simulink model "simltic"  (Simulink 8.5)
settings: Solver=ode45  StartTime=0.0  StopTime=1  RelTol=1e-3
values from neighbouring files (symbols this model uses):
  F = [0  1; -0.9  -0.8]    [harmosc_ricatti.mat]    (also in harmosc_riccati.mat; lec.m = ones(n,1); state9.m = [ 0     rho_z  -rho_y     1     0     0     0     0     0; state9_01.mat = [0 0 -7.85492378154e-07 -1.53754144823e-06 0 0 0 0 0 0 0 -7.)
  H = [1 0]    [constant_velocity.m]    (also in damposc.m; harmosc_ricatti.mat; harmosc_riccati.mat; kf_resistor_demo.m = 1)
  I = [1  0; 0  1]    [harmosc_ricatti.mat]    (also in harmosc_riccati.mat; kalgen.m = eye(n); lec.m = ones(n,1); state9.m = eye(n))
  P0 = [0.01 0; 0 0.01]    [constant_velocity.m]    (also in damposc.m; harmosc_ricatti.mat = [0.95  0; 0  1]; harmosc_riccati.mat = [1  0; 0  1]; kalgen.m = proc_noise * eye(n))
  Q = [0.0001 0; 0 0.000001]    [constant_velocity.m]    (also in damposc.m = [0.00001 0; 0 0.000001]; harmosc_ricatti.mat = [1  0; 0  1]; harmosc_riccati.mat = [1  0; 0  1]; kalgen.m = proc_noise * eye(n))
  R = Re + h    (= 6378441.8)    [Ainit.m]    (also in constant_velocity.m = 1; damposc.m = 0.01; harmosc_ricatti.mat = 2; harmosc_riccati.mat = 3)
undefined symbols (not defined in the file or in its folder): rss_ratio, ud_inv
settings Model: Creator=mcarroll  LastModifiedBy=1104070  ExtModeAutoUpdateStatusClock=off
settings DataIOCC: SaveFormat=StructureWithTime  SignalLoggingName=sigsOut
settings OptimizationCC: OptimizeBlockIOStorage=off  BufferReuse=off  GlobalBufferReuse=off  ExpressionFolding=off  LocalBlockOutputs=off
settings DebuggingCC: SaveWithParameterizedLinksMsg=none  SignalResolutionControl=TryResolveAllWithWarning  MultiTaskDSMMsg=warning  MultiTaskCondExecSysMsg=none  FcnCallInpInsideContextMsg=UseLocalSettings
settings HardwareCC: TargetUnknown=on

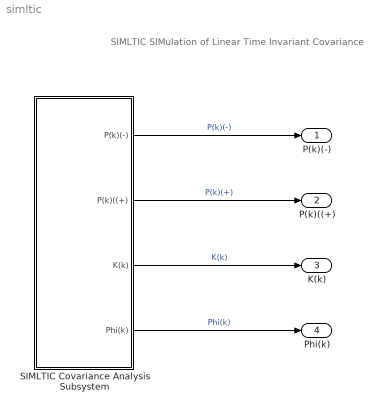
== system simltic ==
  note: SIMLTIC
      | SIMulation of Linear Time Invariant Covariance
  SIMLTIC Covariance Analysis Subsystem : Subsystem
  P(k)(-) : Outport
  P(k)((+) : Outport  Port=2
  K(k) : Outport  Port=3
  Phi(k) : Outport  Port=4
  wires:
  SIMLTIC Covariance Analysis Subsystem/1(P(k)(-)) -> P(k)(-)/1  "P(k)(-)"
  SIMLTIC Covariance Analysis Subsystem/2(P(k)((+)) -> P(k)((+)/1  "P(k)(+)"
  SIMLTIC Covariance Analysis Subsystem/3(K(k)) -> K(k)/1  "K(k)"
  SIMLTIC Covariance Analysis Subsystem/4(Phi(k)) -> Phi(k)/1  "Phi(k)"

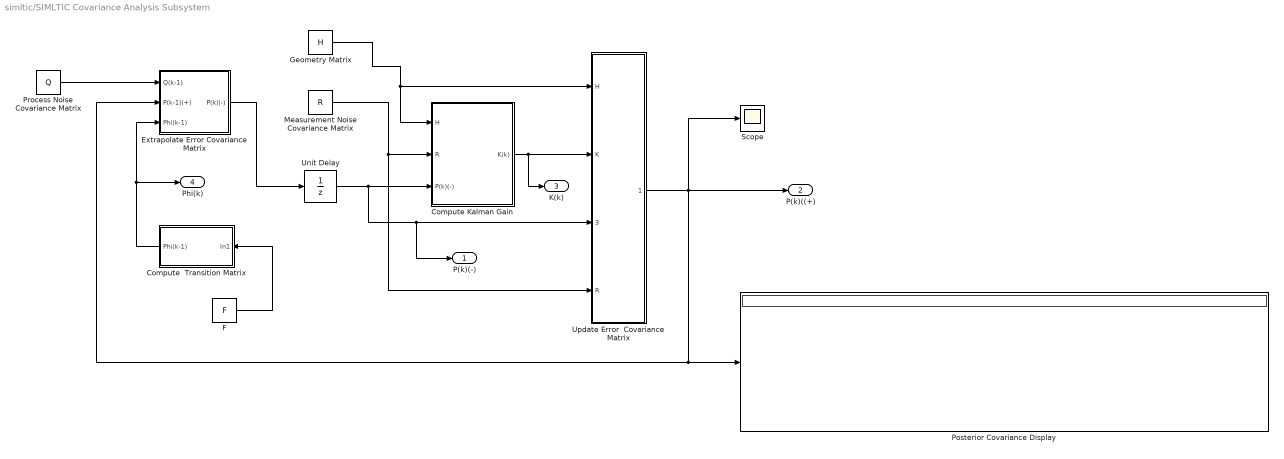
== system simltic/SIMLTIC Covariance Analysis Subsystem ==
  Compute  Transition Matrix : Subsystem
  Compute Kalman Gain : Subsystem
  Extrapolate Error Covariance Matrix : Subsystem
  F : Constant  Value=F  VectorParams1D=off
  Geometry Matrix : Constant  Value=H  VectorParams1D=off
  Measurement Noise Covariance Matrix : Constant  Value=R  VectorParams1D=off
  Posterior Covariance Display : Display
  Process Noise Covariance Matrix : Constant  Value=Q  VectorParams1D=off
  Scope : Scope
      settings: TimeRange=10  YMin=-20  YMax=120  SaveName=ScopeData4
  Unit Delay : UnitDelay  InitialCondition=P0
  Update Error  Covariance Matrix : Subsystem
  P(k)(-) : Outport
  P(k)((+) : Outport  Port=2
  K(k) : Outport  Port=3
  Phi(k) : Outport  Port=4
  wires:
  Update Error  Covariance Matrix/1(P(k)(+)) -> Extrapolate Error Covariance Matrix/2(P(k-1)(+)), Posterior Covariance Display/1, P(k)((+)/1, Scope/1
  Unit Delay/1 -> Compute Kalman Gain/3(P(k)(-)), Update Error  Covariance Matrix/3(P(k)(-)), P(k)(-)/1
  Compute Kalman Gain/1(K(k)) -> Update Error  Covariance Matrix/2(K), K(k)/1
  Process Noise Covariance Matrix/1 -> Extrapolate Error Covariance Matrix/1(Q(k-1))
  Extrapolate Error Covariance Matrix/1(P(k)(-)) -> Unit Delay/1
  Compute  Transition Matrix/1(Phi(k-1)) -> Extrapolate Error Covariance Matrix/3(Phi(k-1)), Phi(k)/1
  Geometry Matrix/1 -> Compute Kalman Gain/1(H), Update Error  Covariance Matrix/1(H)
  Measurement Noise Covariance Matrix/1 -> Compute Kalman Gain/2(R), Update Error  Covariance Matrix/4(R)
  F/1 -> Compute  Transition Matrix/1(In1)

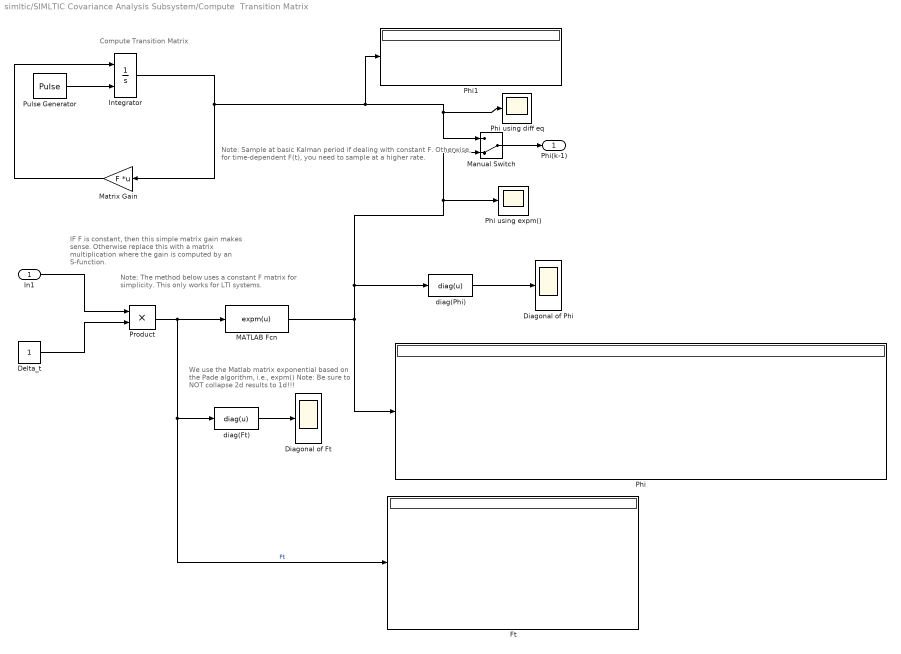
== system simltic/SIMLTIC Covariance Analysis Subsystem/Compute  Transition Matrix ==
  note: We use the Matlab matrix exponential based
      | on the Pade algorithm, i.e., expm()
      | Note:  Be sure to NOT collapse 2d results
      | to 1d!!!
  note: Note:  The method below uses a constant F matrix
      | for simplicity.  This only works for LTI
      | systems.
  note: Compute Transition Matrix
  note: Note: Sample at basic Kalman period if dealing with constant F.
      | Otherwise, for time-dependent F(t), you need to sample at a
      | higher rate.
  note: IF F is constant, then this simple
      | matrix gain makes sense.  Otherwise
      | replace this with a matrix multiplication
      | where the gain is computed by an S-function.
  In1 : Inport
  Delta_t : Constant
  Diagonal of Ft : Scope
      settings: YMin=0  YMax=2  SaveName=ScopeData18
  Diagonal of Phi : Scope
      settings: YMin=0  YMax=2  SaveName=ScopeData3
  Ft : Display
  Integrator : Integrator  ExternalReset=either  InitialCondition=I
  MATLAB Fcn : MATLABFcn  MATLABFcn=expm(u)  Output1D=off
  Manual Switch : ManualSwitch  CurrentSetting=0
  Matrix Gain : Gain  Gain=F  Multiplication=Matrix(K*u)  SaturateOnIntegerOverflow=on  OutDataTypeStr=Inherit: Same as input  ParamDataTypeStr=Inherit: Same as input
  Phi : Display
  Phi using diff eq : Scope
      settings: YMin=0  YMax=2  SaveName=ScopeData11
  Phi using expm() : Scope
      settings: YMin=0  YMax=2  SaveName=ScopeData5
  Phi1 : Display
  Product : Product  SaturateOnIntegerOverflow=on  InputSameDT=on  OutDataTypeStr=Inherit: Same as first input
  Pulse Generator : DiscretePulseGenerator  PulseType=Time based  PulseWidth=50
  diag(Ft) : MATLABFcn  MATLABFcn=diag(u)  Output1D=off
  diag(Phi) : MATLABFcn  MATLABFcn=diag(u)
  Phi(k-1) : Outport
  wires:
  Delta_t/1 -> Product/2
  diag(Ft)/1 -> Diagonal of Ft/1
  diag(Phi)/1 -> Diagonal of Phi/1
  MATLAB Fcn/1 -> Phi/1, diag(Phi)/1, Manual Switch/2, Phi using expm()/1
  Product/1 -> diag(Ft)/1, Ft/1, MATLAB Fcn/1  "Ft"
  In1/1 -> Product/1
  Integrator/1 -> Matrix Gain/1, Phi1/1, Manual Switch/1, Phi using diff eq/1
  Manual Switch/1 -> Phi(k-1)/1
  Matrix Gain/1 -> Integrator/1
  Pulse Generator/1 -> Integrator/2

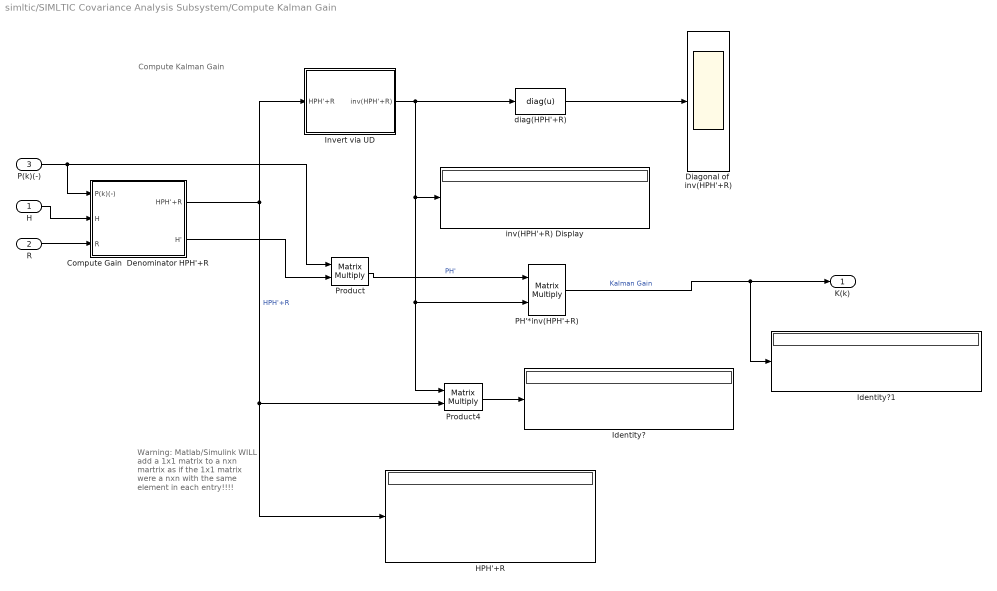
== system simltic/SIMLTIC Covariance Analysis Subsystem/Compute Kalman Gain ==
  note: Compute Kalman Gain
  note: Warning:
      | Matlab/Simulink
      | WILL add a 1x1 matrix to
      | a nxn martrix as if the
      | 1x1 matrix were a
      | nxn with the same element
      | in each entry!!!!
  H : Inport
  R : Inport  Port=2
  P(k)(-) : Inport  Port=3
  Compute Gain  Denominator HPH'+R : Subsystem
  Diagonal of  inv(HPH'+R) : Scope
      settings: TimeRange=100  YMin=0.0006  YMax=0.002  SaveName=ScopeData2
  HPH'+R : Display
  Identity? : Display
  Identity?1 : Display
  Invert via UD : Subsystem
  PH'*inv(HPH'+R) : Product  Multiplication=Matrix(*)  OutDataTypeStr=Inherit: Same as first input
  Product : Product  Multiplication=Matrix(*)  SaturateOnIntegerOverflow=on  OutDataTypeStr=Inherit: Same as first input
  Product4 : Product  Multiplication=Matrix(*)  SaturateOnIntegerOverflow=on  InputSameDT=on  OutDataTypeStr=Inherit: Same as first input
  diag(HPH'+R) : MATLABFcn  MATLABFcn=diag(u)
  inv(HPH'+R) Display : Display
  K(k) : Outport
  wires:
  Compute Gain  Denominator HPH'+R/1(HPH'+R) -> Invert via UD/1(HPH'+R), HPH'+R/1, Product4/2  "HPH'+R"
  R/1 -> Compute Gain  Denominator HPH'+R/3(R)
  diag(HPH'+R)/1 -> Diagonal of  inv(HPH'+R)/1
  Invert via UD/1(inv(HPH'+R)) -> diag(HPH'+R)/1, inv(HPH'+R) Display/1, PH'*inv(HPH'+R)/2, Product4/1
  Compute Gain  Denominator HPH'+R/2(H') -> Product/2
  Product/1 -> PH'*inv(HPH'+R)/1  "PH'"
  Product4/1 -> Identity?/1
  H/1 -> Compute Gain  Denominator HPH'+R/2(H)
  P(k)(-)/1 -> Compute Gain  Denominator HPH'+R/1(P(k)(-)), Product/1
  PH'*inv(HPH'+R)/1 -> K(k)/1, Identity?1/1  "Kalman Gain"

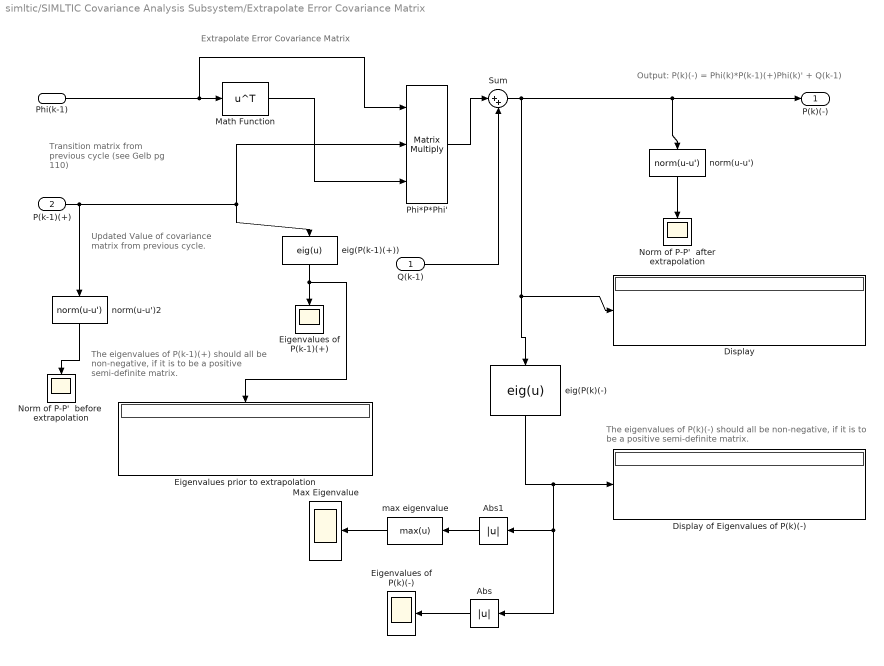
== system simltic/SIMLTIC Covariance Analysis Subsystem/Extrapolate Error Covariance Matrix ==
  note: The eigenvalues of P(k)(-) should all be non-negative,
      | if it is to be a positive semi-definite matrix.
  note: The eigenvalues of P(k-1)(+) should all be
      | non-negative, if it is to be a positive
      | semi-definite matrix.
  note: Transition matrix from
      | previous cycle
      | (see Gelb pg 110)
  note: Output: P(k)(-) = Phi(k)*P(k-1)(+)Phi(k)' + Q(k-1)
  note: Updated Value of
      | covariance matrix  from
      | previous cycle.
  note: Extrapolate Error Covariance Matrix
  Q(k-1) : Inport
  P(k-1)(+) : Inport  Port=2
  Phi(k-1) : Inport  Port=3
  Abs : Abs  SaturateOnIntegerOverflow=on
  Abs1 : Abs  SaturateOnIntegerOverflow=on
  Display : Display
  Display of Eigenvalues of P(k)(-) : Display
  Eigenvalues prior to extrapolation : Display
  Eigenvalues of P(k)(-) : Scope
      settings: SaveName=ScopeData8
  Eigenvalues of P(k-1)(+) : Scope
      settings: YMin=1  YMax=8.5  SaveName=ScopeData7
  Math Function : Math  Operator=transpose  SaturateOnIntegerOverflow=on
  Max Eigenvalue : Scope
      settings: TimeRange=100  YMin=0  YMax=4e+072  SaveName=ScopeData12
  Norm of P-P'  after extrapolation : Scope
      settings: TimeRange=10  YMin=0  YMax=35  SaveName=ScopeData15
  Norm of P-P'  before  extrapolation : Scope
      settings: TimeRange=10  YMin=0  YMax=35  SaveName=ScopeData16
  Phi*P*Phi' : Product  Inputs=3  Multiplication=Matrix(*)  SaturateOnIntegerOverflow=on  InputSameDT=on  OutDataTypeStr=Inherit: Same as first input
  Sum : Sum  Inputs=|++  SaturateOnIntegerOverflow=on  InputSameDT=on  OutDataTypeStr=Inherit: Same as first input
  eig(P(k)(-) : MATLABFcn  MATLABFcn=eig(u)  OutputSignalType=complex
  eig(P(k-1)(+)) : MATLABFcn  MATLABFcn=eig(u)
  max eigenvalue : MATLABFcn  MATLABFcn=max(u)  Output1D=off
  norm(u-u') : MATLABFcn  MATLABFcn=norm(u-u')  Output1D=off
  norm(u-u')2 : MATLABFcn  MATLABFcn=norm(u-u')  Output1D=off
  P(k)(-) : Outport
  wires:
  Math Function/1 -> Phi*P*Phi'/3
  max eigenvalue/1 -> Max Eigenvalue/1
  Abs1/1 -> max eigenvalue/1
  Abs/1 -> Eigenvalues of P(k)(-)/1
  norm(u-u')2/1 -> Norm of P-P'  before  extrapolation/1
  norm(u-u')/1 -> Norm of P-P'  after extrapolation/1
  eig(P(k)(-)/1 -> Display of Eigenvalues of P(k)(-)/1, Abs1/1, Abs/1
  eig(P(k-1)(+))/1 -> Eigenvalues prior to extrapolation/1, Eigenvalues of P(k-1)(+)/1
  Q(k-1)/1 -> Sum/2
  P(k-1)(+)/1 -> Phi*P*Phi'/2, eig(P(k-1)(+))/1, norm(u-u')2/1
  Phi(k-1)/1 -> Phi*P*Phi'/1, Math Function/1
  Sum/1 -> norm(u-u')/1, P(k)(-)/1, eig(P(k)(-)/1, Display/1
  Phi*P*Phi'/1 -> Sum/1

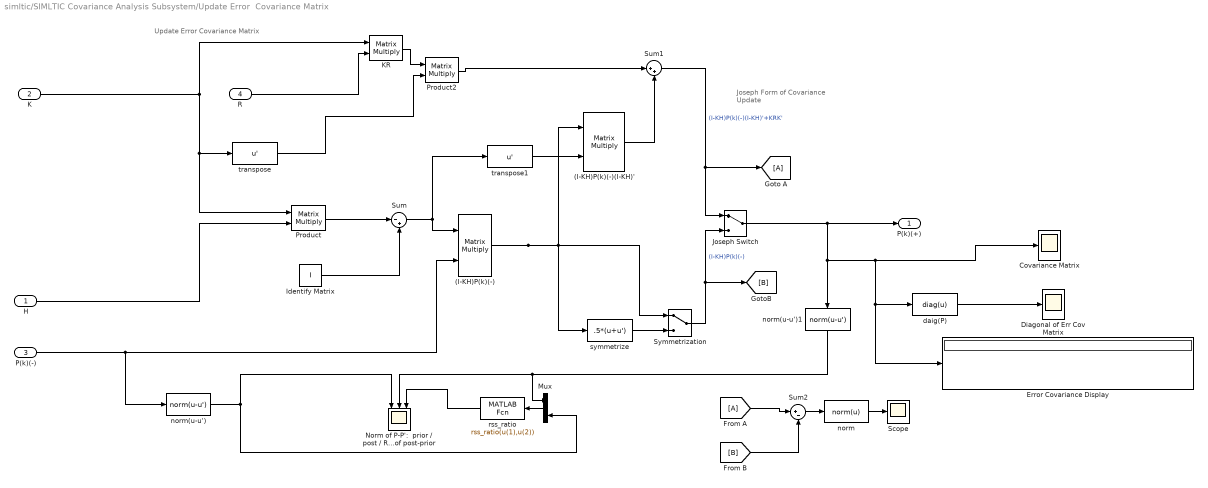
== system simltic/SIMLTIC Covariance Analysis Subsystem/Update Error  Covariance Matrix ==
  note: Update Error Covariance Matrix
  note: Joseph Form
      | of Covariance
      | Update
  H : Inport
  K : Inport  Port=2
  P(k)(-) : Inport  Port=3
  R : Inport  Port=4
  (I-KH)P(k)(-) : Product  Multiplication=Matrix(*)  SaturateOnIntegerOverflow=on  InputSameDT=on  OutDataTypeStr=Inherit: Same as first input
  (I-KH)P(k)(-)(I-KH)' : Product  Multiplication=Matrix(*)  SaturateOnIntegerOverflow=on  InputSameDT=on  OutDataTypeStr=Inherit: Same as first input
  Covariance Matrix : Scope
      settings: TimeRange=10  YMin=-60  YMax=80
  Diagonal of Err Cov Matrix : Scope
      settings: YMin=0  YMax=5000
  Error Covariance Display : Display
  Identify Matrix : Constant  Value=I  VectorParams1D=off
  Joseph Switch : ManualSwitch
  KR : Product  Multiplication=Matrix(*)  SaturateOnIntegerOverflow=on  OutDataTypeStr=Inherit: Same as first input
  Mux : Mux  Inputs=2
  Norm of P-P':  prior / post / RSS ratio of post-prior : Scope  NumInputPorts=3
      settings: TimeRange=10  YMin=0~0~0  YMax=40~2~0.05  SaveName=ScopeData13
  Product : Product  Multiplication=Matrix(*)  SaturateOnIntegerOverflow=on  InputSameDT=on  OutDataTypeStr=Inherit: Same as first input
  Product2 : Product  Multiplication=Matrix(*)  SaturateOnIntegerOverflow=on  OutDataTypeStr=Inherit: Same as first input
  Scope : Scope
      settings: SaveName=ScopeData14
  Sum : Sum  Inputs=|-+  SaturateOnIntegerOverflow=on  InputSameDT=on  OutDataTypeStr=Inherit: Same as first input
  Sum1 : Sum  Inputs=|++  SaturateOnIntegerOverflow=on  InputSameDT=on  OutDataTypeStr=Inherit: Same as first input
  Sum2 : Sum  Inputs=|+-  SaturateOnIntegerOverflow=on  InputSameDT=on  OutDataTypeStr=Inherit: Same as first input
  Symmetrization : ManualSwitch
  daig(P) : MATLABFcn  MATLABFcn=diag(u)
  norm : MATLABFcn  MATLABFcn=norm(u)  Output1D=off
  norm(u-u') : MATLABFcn  MATLABFcn=norm(u-u')  Output1D=off
  norm(u-u')1 : MATLABFcn  MATLABFcn=norm(u-u')  Output1D=off
  rss_ratio : MATLABFcn  MATLABFcn=rss_ratio(u(1),u(2))  OutputSignalType=real
  symmetrize : MATLABFcn  MATLABFcn=.5*(u+u')  Output1D=off
  transpose : MATLABFcn  MATLABFcn=u'  Output1D=off
  transpose1 : MATLABFcn  MATLABFcn=u'  Output1D=off
  P(k)(+) : Outport
  wires:
  H/1 -> Product/2
  K/1 -> Product/1, transpose/1, KR/1
  P(k)(-)/1 -> (I-KH)P(k)(-)/2, norm(u-u')/1
  Identify Matrix/1 -> Sum/2
  Product/1 -> Sum/1
  Sum/1 -> (I-KH)P(k)(-)/1, transpose1/1
  R/1 -> KR/2
  transpose/1 -> Product2/2
  (I-KH)P(k)(-)/1 -> (I-KH)P(k)(-)(I-KH)'/1, Symmetrization/1, symmetrize/1
  transpose1/1 -> (I-KH)P(k)(-)(I-KH)'/2
  (I-KH)P(k)(-)(I-KH)'/1 -> Sum1/2
  Product2/1 -> Sum1/1
  symmetrize/1 -> Symmetrization/2
  Symmetrization/1 -> Joseph Switch/2, [B]  "(I-KH)P(k)(-)"
  Joseph Switch/1 -> P(k)(+)/1, norm(u-u')1/1, daig(P)/1, Error Covariance Display/1, Covariance Matrix/1
  Sum1/1 -> Joseph Switch/1, [A]  "(I-KH)P(k)(-)(I-KH)'+KRK'"
  norm(u-u')/1 -> Norm of P-P':  prior / post / RSS ratio of post-prior/1, Mux/2
  norm(u-u')1/1 -> Norm of P-P':  prior / post / RSS ratio of post-prior/2, Mux/1
  rss_ratio/1 -> Norm of P-P':  prior / post / RSS ratio of post-prior/3
  Mux/1 -> rss_ratio/1
  [B] -> Sum2/2
  [A] -> Sum2/1
  Sum2/1 -> norm/1
  norm/1 -> Scope/1
  daig(P)/1 -> Diagonal of Err Cov Matrix/1
  KR/1 -> Product2/1

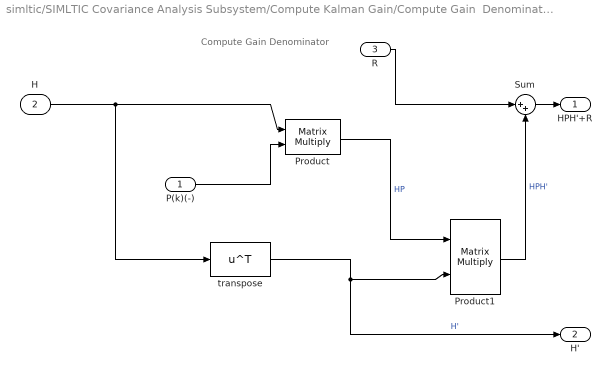
== system simltic/SIMLTIC Covariance Analysis Subsystem/Compute Kalman Gain/Compute Gain  Denominator HPH'+R ==
  note: Compute Gain Denominator
  P(k)(-) : Inport
  H : Inport  Port=2
  R : Inport  Port=3
  Product : Product  Multiplication=Matrix(*)  SaturateOnIntegerOverflow=on  InputSameDT=on  OutDataTypeStr=Inherit: Same as first input
  Product1 : Product  Multiplication=Matrix(*)  SaturateOnIntegerOverflow=on  InputSameDT=on  OutDataTypeStr=Inherit: Same as first input
  Sum : Sum  Inputs=|++  SaturateOnIntegerOverflow=on  InputSameDT=on  OutDataTypeStr=Inherit: Same as first input
  transpose : Math  Operator=transpose  SaturateOnIntegerOverflow=on
  HPH'+R : Outport
  H' : Outport  Port=2
  wires:
  transpose/1 -> H'/1, Product1/2  "H'"
  Product1/1 -> Sum/2  "HPH'"
  Product/1 -> Product1/1  "HP"
  H/1 -> Product/1, transpose/1
  R/1 -> Sum/1
  Sum/1 -> HPH'+R/1
  P(k)(-)/1 -> Product/2

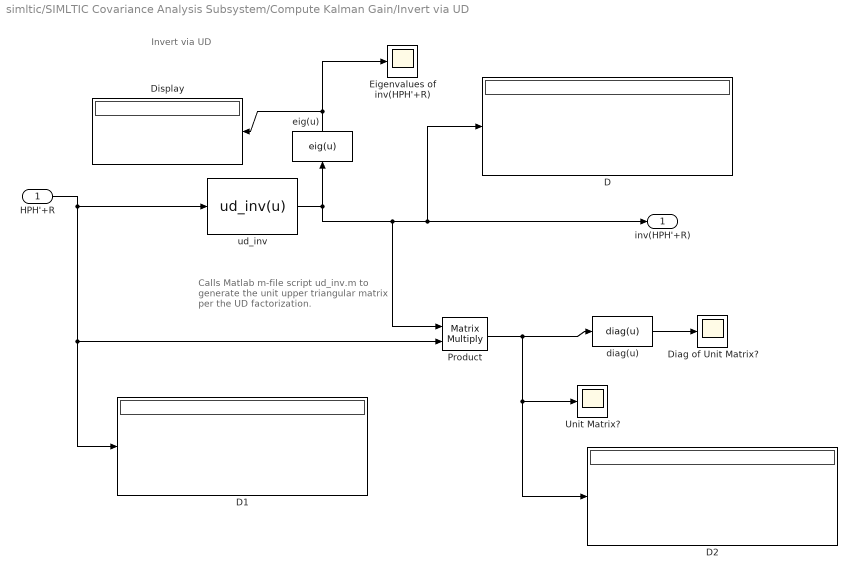
== system simltic/SIMLTIC Covariance Analysis Subsystem/Compute Kalman Gain/Invert via UD ==
  note: Calls Matlab m-file script ud_inv.m
      | to generate the unit upper triangular
      | matrix per the UD factorization.
  note: Invert via UD
  HPH'+R : Inport
  D : Display
  D1 : Display
  D2 : Display
  Diag of Unit Matrix? : Scope
      settings: YMin=0.99  YMax=1.03  SaveName=ScopeData10
  Display : Display
  Eigenvalues of inv(HPH'+R) : Scope
      settings: SaveName=ScopeData6
  Product : Product  Multiplication=Matrix(*)  SaturateOnIntegerOverflow=on  InputSameDT=on  OutDataTypeStr=Inherit: Same as first input
  Unit Matrix? : Scope
      settings: SaveName=ScopeData9
  diag(u) : MATLABFcn  MATLABFcn=diag(u)  Output1D=off
  eig(u) : MATLABFcn  MATLABFcn=eig(u)  Output1D=off
  ud_inv : MATLABFcn  MATLABFcn=ud_inv(u)  Output1D=off
  inv(HPH'+R) : Outport
  wires:
  HPH'+R/1 -> ud_inv/1, D1/1, Product/2
  ud_inv/1 -> eig(u)/1, inv(HPH'+R)/1, D/1, Product/1
  eig(u)/1 -> Eigenvalues of inv(HPH'+R)/1, Display/1
  Product/1 -> diag(u)/1, Unit Matrix?/1, D2/1
  diag(u)/1 -> Diag of Unit Matrix?/1
